simulink model "shiftcontroller"  (R2024b)
settings: Solver=VariableStepAuto  StartTime=0.0  StopTime=1e-5  RelTol=1e-3
undefined symbols (not defined in the file): plecs
settings Model: Creator=Goat_  LastModifiedBy=Goat_

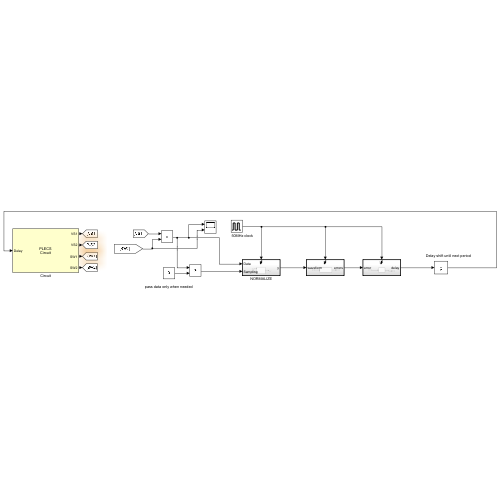
[thumbnail: Simulink's stored preview of the top-level diagram]
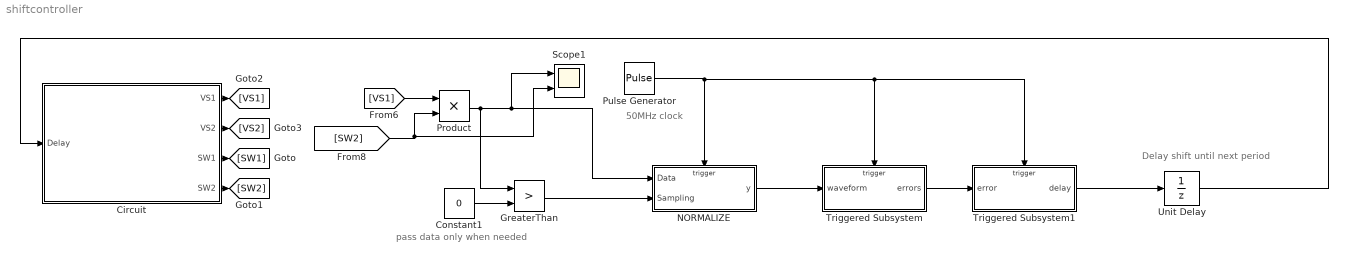
== system shiftcontroller ==
  note: Delay shift until next period
  note: 50MHz clock
  note: pass data only when needed
  Circuit : Subsystem  LoadFcn=plecs('sl', 200);  InitFcn=plecs('sl', 214);  StartFcn=plecs('sl', 208);  StopFcn=plecs('sl', 209);  mask(PlecsCircuit){PLECSData=<binary blob, 10052 chars, not shown>}
      mask prompts: PLECSData "PLECS Data (Do not delete or modify!)"
      mask init:
      | % PLACE CUSTOM INITIALIZATIONS ABOVE
      | % DO NOT REMOVE
      | plecs('sl', 215);
      | % DO NOT REMOVE
      settings: CopyFcn=plecs('sl', 203);  DeleteFcn=plecs('sl', 205);  UndoDeleteFcn=plecs('sl', 206);  PreSaveFcn=plecs('sl', 211);  PostSaveFcn=plecs('sl', 201);  NameChangeFcn=plecs('sl', 210);  DestroyFcn=plecs('sl', 207);  PreCopyFcn=plecs('sl', 216);  OpenFcn=plecs('sl', 202);  ErrorFcn=plerrorfcn
      mask Help: eval('plecs(''help'', ''qthelp:///creatingacircuit.html'')')
      mask Display: disp('PLECS\nCircuit')
  Constant1 : Constant  Value=0
  GreaterThan : RelationalOperator  Operator=>  OutDataTypeStr=boolean  RndMeth=Simplest  InputSameDT=off
  NORMALIZE : Subsystem  TreatAsAtomicUnit=on
  Product : Product
  Pulse Generator : DiscretePulseGenerator  PulseType=Time based  Period=1/(50e6)  PulseWidth=5
  Scope1 : Scope  NumInputPorts=2
  Triggered Subsystem : Subsystem  TreatAsAtomicUnit=on
  Triggered Subsystem1 : Subsystem  TreatAsAtomicUnit=on
  Unit Delay : UnitDelay  SampleTime=1/(10e6)  HasFrameUpgradeWarning=on
  wires:
  Circuit/1(VS1) -> [VS1]
  Circuit/2(VS2) -> [VS2]
  Circuit/3(SW1) -> [SW1]
  Circuit/4(SW2) -> [SW2]
  [VS1] -> Product/1
  Product/1 -> Scope1/1, NORMALIZE/1(Data), GreaterThan/1
  [SW2] -> Scope1/2, Product/2
  Constant1/1 -> GreaterThan/2
  Pulse Generator/1 -> Triggered Subsystem1/Trigger, Triggered Subsystem/Trigger, NORMALIZE/Trigger
  GreaterThan/1 -> NORMALIZE/2(Sampling)
  NORMALIZE/1(y) -> Triggered Subsystem/1(waveform)
  Unit Delay/1 -> Circuit/1(Delay)
  Triggered Subsystem1/1(delay) -> Unit Delay/1
  Triggered Subsystem/1(errors) -> Triggered Subsystem1/1(error)

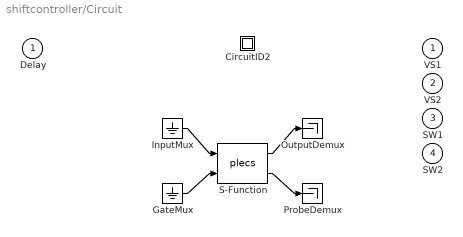
== system shiftcontroller/Circuit ==
  Delay : Inport  PortDimensions=1
  " CircuitID2 " : Subsystem
  " GateMux " : Ground
  " InputMux " : Ground
  " OutputDemux " : Terminator
  " ProbeDemux " : Terminator
  " S-Function " : S-Function  FunctionName=plecs  SFunctionDeploymentMode=off  EnableBusSupport=off
  VS1 : Outport  PortDimensions=1
  VS2 : Outport  Port=2  PortDimensions=1
  SW1 : Outport  Port=3  PortDimensions=1
  SW2 : Outport  Port=4  PortDimensions=1
  wires:
  " InputMux "/1 -> " S-Function "/1
  " GateMux "/1 -> " S-Function "/2
  " S-Function "/1 -> " OutputDemux "/1
  " S-Function "/2 -> " ProbeDemux "/1

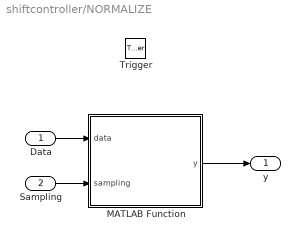
== system shiftcontroller/NORMALIZE ==
  Data : Inport
  Sampling : Inport  Port=2
  Trigger : TriggerPort  VariantControl=(inherit)
  MATLAB Function : MATLAB Function  TreatAsAtomicUnit=on
  y : Outport
  wires:
  Sampling/1 -> MATLAB Function/2(sampling)
  Data/1 -> MATLAB Function/1(data)
  MATLAB Function/1(y) -> y/1

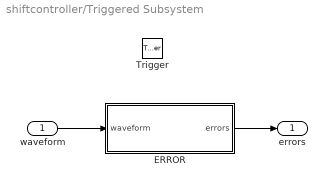
== system shiftcontroller/Triggered Subsystem ==
  waveform : Inport
  Trigger : TriggerPort  VariantControl=(inherit)
  ERROR : MATLAB Function  TreatAsAtomicUnit=on
  errors : Outport
  wires:
  waveform/1 -> ERROR/1(waveform)
  ERROR/1(errors) -> errors/1

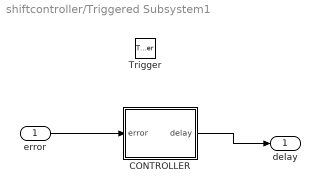
== system shiftcontroller/Triggered Subsystem1 ==
  error : Inport
  Trigger : TriggerPort  VariantControl=(inherit)
  CONTROLLER : MATLAB Function  TreatAsAtomicUnit=on
  delay : Outport
  wires:
  error/1 -> CONTROLLER/1(error)
  CONTROLLER/1(delay) -> delay/1

== system shiftcontroller/Circuit/ CircuitID2  ==

== matlab function shiftcontroller/NORMALIZE/MATLAB Function ==
  data: data input; y output; sampling input
function y = fcn(data, sampling)
persistent semisample idx

if isempty(semisample)
    semisample = zeros(1, 50);
end
if isempty(idx)
    idx = 1;
end

y = zeros(1,50);

if sampling %So long as sampling a pulse
    if idx <= length(semisample)
        semisample(idx) = data;
        idx = idx + 1;
    end
end

if ~sampling && ~all(semisample==0) %Send data when stop sampling
    m = max(semisample);
    semisample = semisample/m;
    y = semisample;
    semisample = zeros(1, 50);
    idx = 1;
elseif ~sampling
    y = zeros(1,50);
end

% if ~all(y==0)
%     disp(y);
% end

== matlab function shiftcontroller/Triggered Subsystem1/CONTROLLER ==
  data: error input; delay output
function delay = fcn(error)

y = 0;
delay = 0;

if ~all(error==0)
    clipped_error = error(error ~= 0);
    phase_shift = clipped_error(length(clipped_error));
    
    k = -1;
    
    delay = 1 + (k * phase_shift);
    % delay = (1+y)/(10e6);
    disp(delay);
    
end

== matlab function shiftcontroller/Triggered Subsystem/ERROR ==
  data: waveform input; errors output
function errors = fcn(waveform)

wave_clipped = nonzeros(waveform);
sineref = zeros(1,50);
errors = zeros(1,50);

if ~all(waveform==0)
    for i = 1:1:length(wave_clipped)
        if(i<=length(wave_clipped))
            sineref(i) = sin(pi*i/length(wave_clipped));
        end
    end
    
    errors = waveform-sineref;

    %disp(errors);
end
